simulink model "Simulacion_Trifasico_Fuzzy_v10_v12"  (R2024a)
settings: Solver=ode3  StartTime=0  StopTime=tend  FixedStep=0.01  RelTol=1e-3
values from neighbouring files (symbols this model uses):
  ts = 0.1    [Fuzzy_init.m]    (also in MPC_linealizar_v6.m)
libraries: simulink x6, eeStairGenerator x6, fuzblock x1
settings Model: Creator=Ivan  LastModifiedBy=Ivan
settings DebuggingCC: UnderSpecifiedDimensionMsg=warning
settings ConfigComp: PLC_TargetIDE=tiaportal  PLC_MultiTBSigbuilderTimeRange=off  PLC_FoldFBCallOutputVar=off  PLC_RemoveUnusedSSMethodCallArguments=off  PLC_UseCallOutputArgSyntax=off  PLC_EnableUnsignedAndDoubleTypes=off  PLC_EnableUDTSplitting=off  PLC_MaxFieldsInUDT=500  PLC_InlineEnumCastFunction=off

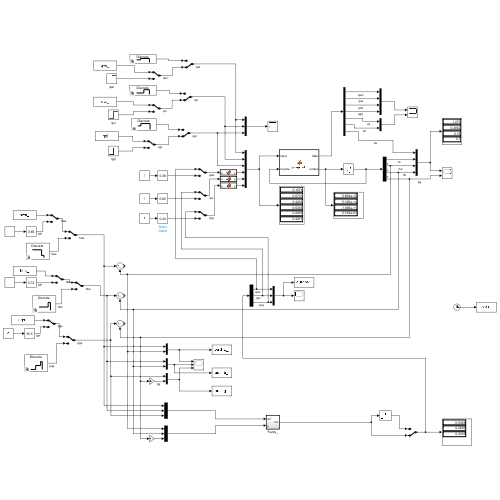
[thumbnail: Simulink's stored preview of the top-level diagram]
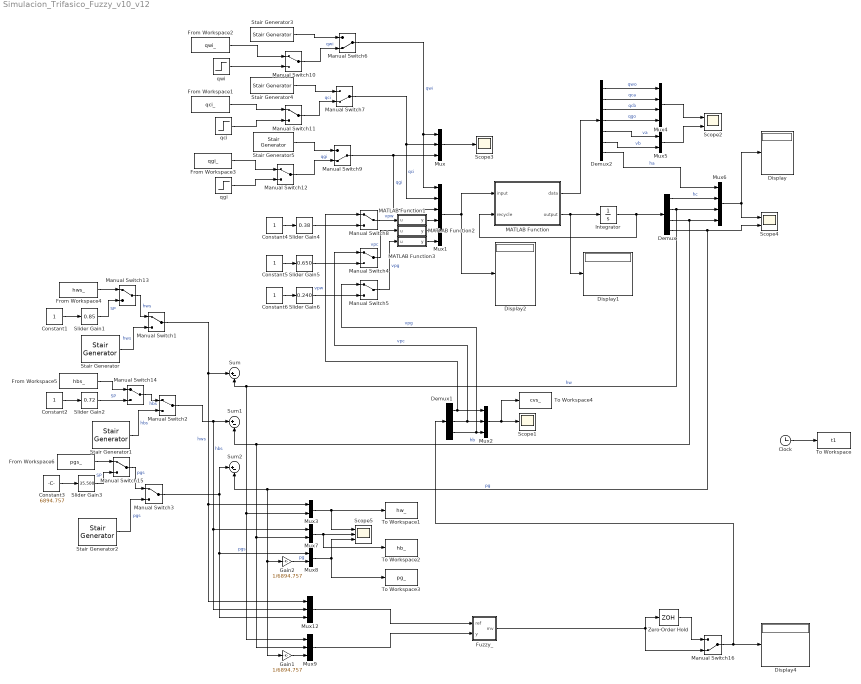
== system Simulacion_Trifasico_Fuzzy_v10_v12 ==
  Clock : Clock
  Constant{1..2,4..6} (5 alike) : Constant
  Constant3 : Constant  Value=6894.757
  Demux : Demux
  Demux1 : Demux  Outputs=3
  Demux2 : Demux  Outputs=7
  Display{,1..2,4} (4 alike) : Display
  From Workspace1 : FromWorkspace  VariableName=qci_  SampleTime=ts
  From Workspace2 : FromWorkspace  VariableName=qwi_  SampleTime=ts
  From Workspace3 : FromWorkspace  VariableName=qgi_  SampleTime=ts
  From Workspace4 : FromWorkspace  VariableName=hws_  SampleTime=ts
  From Workspace5 : FromWorkspace  VariableName=hbs_  SampleTime=ts
  From Workspace6 : FromWorkspace  VariableName=pgs_  SampleTime=ts
  Fuzzy_ : Subsystem  TreatAsAtomicUnit=on  SystemSampleTime=0.1
  Gain1 : Gain  Gain=1/6894.757
  Gain2 : Gain  Gain=1/6894.757
  Integrator : Integrator  InitialCondition=[0.4737; 0.80; 0.72; 37*6894.757]  LimitOutput=on  LowerSaturationLimit=0
  MATLAB Function : MATLAB Function  TreatAsAtomicUnit=on
  MATLAB Function1 : MATLAB Function  TreatAsAtomicUnit=on
  MATLAB Function2 : MATLAB Function  TreatAsAtomicUnit=on
  MATLAB Function3 : MATLAB Function  TreatAsAtomicUnit=on
  Manual Switch{1..5,8,10..15} (12 alike) : ManualSwitch
  Manual Switch{6..7,9,16} (4 alike) : ManualSwitch  CurrentSetting=0
  Mux{,2,9,12} (4 alike) : Mux  Inputs=3
  Mux1 : Mux  Inputs=6
  Mux{3,5,7..8} (4 alike) : Mux  Inputs=2
  Mux4 : Mux
  Mux6 : Mux
  Scope1 : Scope
  Scope2 : Scope  NumInputPorts=2
  Scope3 : Scope
  Scope4 : Scope  NumInputPorts=2
  Scope5 : Scope  NumInputPorts=3
  Slider Gain1 : simulink/Math Operations/Slider Gain  gain=0.85  low=0  high=1
  Slider Gain2 : simulink/Math Operations/Slider Gain  gain=0.72  low=0  high=1
  Slider Gain3 : simulink/Math Operations/Slider Gain  gain=35.500  low=0  high=50
  Slider Gain4 : simulink/Math Operations/Slider Gain  gain=0.38  low=0  high=1
  Slider Gain5 : simulink/Math Operations/Slider Gain  gain=0.650  low=0  high=1
  Slider Gain6 : simulink/Math Operations/Slider Gain  gain=0.240  low=0  high=1
  Stair Generator : eeStairGenerator/Stair Generator  LabelModeActiveChoice=Discrete  TimeInput=[0 2000 2500]  AmplitudeInput=[0.85 0.80 0.78]  SampleTime=0.01  RepeatPattern=off  OutDataTypeStr=double
      settings: LibrarySourceBlock=ee_sl_lib/General Control/Stair Generator
  Stair Generator1 : eeStairGenerator/Stair Generator  LabelModeActiveChoice=Discrete  TimeInput=[0 2250 2750]  AmplitudeInput=[0.72 0.75 0.70]  SampleTime=0.01  RepeatPattern=off  OutDataTypeStr=double
      settings: LibrarySourceBlock=ee_sl_lib/General Control/Stair Generator
  Stair Generator2 : eeStairGenerator/Stair Generator  LabelModeActiveChoice=Discrete  TimeInput="[0 1500 3000  3500]"  AmplitudeInput=[35 40 45 35]*6894.757  SampleTime=0.01  RepeatPattern=off  OutDataTypeStr=double
      settings: LibrarySourceBlock=ee_sl_lib/General Control/Stair Generator
  Stair Generator3 : eeStairGenerator/Stair Generator  LabelModeActiveChoice=Discrete  TimeInput=[0 1000 3250]  AmplitudeInput=[0.1374 0.1774 0.0474]  SampleTime=0.01  RepeatPattern=off  OutDataTypeStr=double
      settings: LibrarySourceBlock=ee_sl_lib/General Control/Stair Generator
  Stair Generator4 : eeStairGenerator/Stair Generator  LabelModeActiveChoice=Discrete  TimeInput=[0 1750 3100]  AmplitudeInput=[0.0711 0.1815 0.0298]  SampleTime=0.01  RepeatPattern=off  OutDataTypeStr=double
      settings: LibrarySourceBlock=ee_sl_lib/General Control/Stair Generator
  Stair Generator5 : eeStairGenerator/Stair Generator  LabelModeActiveChoice=Discrete  TimeInput=[0 1000 3750]  AmplitudeInput=[0.4906 0.79606 0.006]  SampleTime=0.01  RepeatPattern=off  OutDataTypeStr=double
      settings: LibrarySourceBlock=ee_sl_lib/General Control/Stair Generator
  Sum : Sum  Inputs=|+-
  Sum1 : Sum  Inputs=|+-
  Sum2 : Sum  Inputs=|+-
  To Workspace : ToWorkspace  VariableName=t1  SampleTime=0.1
  To Workspace1 : ToWorkspace  VariableName=hw_  SampleTime=0.1
  To Workspace2 : ToWorkspace  VariableName=hb_  SampleTime=0.1
  To Workspace3 : ToWorkspace  VariableName=pg_  SampleTime=0.1
  To Workspace4 : ToWorkspace  VariableName=cvs_  SampleTime=0.1
  Zero-Order Hold : ZeroOrderHold  SampleTime=-1
  qci : Step  After=.0711  SampleTime=0
  qgi : Step  After=.4906  SampleTime=0
  qwi : Step  After=.1374  SampleTime=0
  wires:
  Mux/1 -> Scope3/1
  Mux2/1 -> To Workspace4/1, Scope1/1
  Demux2/1 -> Mux4/1  "qwo"
  Demux2/2 -> Mux4/2  "qca"
  Demux2/3 -> Mux4/3  "qcb"
  Demux2/4 -> Mux4/4  "qgo"
  Demux2/5 -> Mux5/1  "va"
  Demux2/6 -> Mux5/2  "vb"
  Mux4/1 -> Scope2/1
  Mux5/1 -> Scope2/2
  Demux2/7 -> Mux6/1  "ha"
  Integrator/1 -> MATLAB Function/2(recycle), Demux/1
  Demux/1 -> Mux6/2  "hc"
  Demux/2 -> Mux9/1, Mux3/2, Sum/2, Mux6/3  "hw"
  Demux/3 -> Mux6/4, Mux9/2, Mux7/2, Sum1/2  "hb"
  Mux6/1 -> Display/1, Scope4/1
  Demux/4 -> Scope4/2, Gain1/1, Gain2/1, Sum2/2  "pg"
  Mux1/1 -> MATLAB Function/1(input), Display2/1
  MATLAB Function/2(output) -> Display1/1, Integrator/1
  MATLAB Function/1(data) -> Demux2/1
  Mux3/1 -> Scope5/1, To Workspace1/1
  Mux7/1 -> To Workspace2/1, Scope5/2
  Mux8/1 -> To Workspace3/1, Scope5/3
  Constant1/1 -> Slider Gain1/1
  Manual Switch1/1 -> Sum/1, Mux12/1, Mux3/1  "hws"
  Stair Generator/1 -> Manual Switch1/2  "hws"
  Constant2/1 -> Slider Gain2/1
  Manual Switch2/1 -> Mux7/1, Mux12/2, Sum1/1  "hbs"
  Constant3/1 -> Slider Gain3/1
  Manual Switch3/1 -> Sum2/1, Mux12/3, Mux8/1  "pgs"
  Stair Generator1/1 -> Manual Switch2/2  "hbs"
  Stair Generator2/1 -> Manual Switch3/2  "pgs"
  Constant4/1 -> Slider Gain4/1
  Slider Gain4/1 -> Manual Switch8/2
  Slider Gain5/1 -> Manual Switch4/2
  Constant5/1 -> Slider Gain5/1
  Slider Gain6/1 -> Manual Switch5/2
  Constant6/1 -> Slider Gain6/1
  Stair Generator3/1 -> Manual Switch6/1
  Stair Generator4/1 -> Manual Switch7/1
  Stair Generator5/1 -> Manual Switch9/1
  Manual Switch6/1 -> Mux1/1, Mux/1  "qwi"
  Manual Switch7/1 -> Mux/2, Mux1/2  "qci"
  Manual Switch9/1 -> Mux/3, Mux1/3  "qgi"
  Clock/1 -> To Workspace/1
  qwi/1 -> Manual Switch10/2
  Manual Switch10/1 -> Manual Switch6/2  "qwi"
  From Workspace2/1 -> Manual Switch10/1
  qci/1 -> Manual Switch11/2
  Manual Switch11/1 -> Manual Switch7/2  "qci"
  From Workspace1/1 -> Manual Switch11/1
  qgi/1 -> Manual Switch12/2
  Manual Switch12/1 -> Manual Switch9/2  "qgi"
  From Workspace3/1 -> Manual Switch12/1
  Slider Gain1/1 -> Manual Switch13/2  "SP"
  Manual Switch13/1 -> Manual Switch1/1  "hws"
  Slider Gain2/1 -> Manual Switch14/2  "SP"
  Manual Switch14/1 -> Manual Switch2/1  "hbs"
  Manual Switch15/1 -> Manual Switch3/1  "pgs"
  Slider Gain3/1 -> Manual Switch15/2  "SP"
  From Workspace4/1 -> Manual Switch13/1
  From Workspace5/1 -> Manual Switch14/1
  From Workspace6/1 -> Manual Switch15/1
  Manual Switch5/1 -> MATLAB Function3/1(u)  "vpg"
  Manual Switch4/1 -> MATLAB Function2/1(u)  "vpc"
  Manual Switch8/1 -> MATLAB Function1/1(u)  "vpw"
  MATLAB Function1/1(y) -> Mux1/4
  MATLAB Function2/1(y) -> Mux1/5
  MATLAB Function3/1(y) -> Mux1/6
  Gain1/1 -> Mux9/3
  Demux1/1 -> Manual Switch8/1, Mux2/1  "vpw"
  Demux1/2 -> Manual Switch4/1, Mux2/2  "vpc"
  Demux1/3 -> Mux2/3, Manual Switch5/1  "vpg"
  Gain2/1 -> Mux8/2  "pg"
  Zero-Order Hold/1 -> Manual Switch16/1
  Manual Switch16/1 -> Demux1/1, Display4/1
  Fuzzy_/1(mv) -> Manual Switch16/2, Zero-Order Hold/1
  Mux12/1 -> Fuzzy_/1(ref)
  Mux9/1 -> Fuzzy_/2(y)

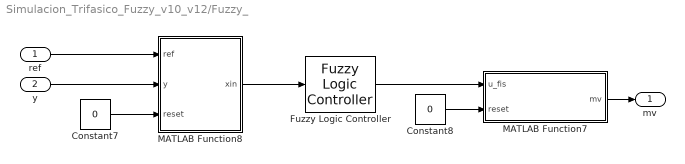
== system Simulacion_Trifasico_Fuzzy_v10_v12/Fuzzy_ ==
  ref : Inport
  y : Inport  Port=2
  Constant7 : Constant  Value=0
  Constant8 : Constant  Value=0
  Fuzzy Logic Controller : fuzblock/Fuzzy Logic  Controller  FIS=fis_tpsep_1block  OutputSampleNumber=101  DataType=double  FuzzifiedInputs=off  RuleFiringStrengths=off  RuleOutputs=off  AggregatedOutputs=off  SimulateUsing=Interpreted execution  OutOfRangeInputValueMessage=warning  NoRuleFiredMessage=warning  EmptyOutputFuzzySetMessage=warning
  MATLAB Function7 : MATLAB Function  TreatAsAtomicUnit=on
  MATLAB Function8 : MATLAB Function  TreatAsAtomicUnit=on
  mv : Outport
  wires:
  ref/1 -> MATLAB Function8/1(ref)
  Constant7/1 -> MATLAB Function8/3(reset)
  MATLAB Function8/1(xin) -> Fuzzy Logic Controller/1
  Fuzzy Logic Controller/1 -> MATLAB Function7/1(u_fis)
  Constant8/1 -> MATLAB Function7/2(reset)
  MATLAB Function7/1(mv) -> mv/1
  y/1 -> MATLAB Function8/2(y)

== matlab function Simulacion_Trifasico_Fuzzy_v10_v12/MATLAB Function ==
  data: input input size=6; data output size=7; output output size=4; recycle input size=4
function [data, output] = tpsep_v12(input, recycle)
%#codegen
% Codigo del bloque MATLAB Function de la planta, version corregida (tpsep_v12).
% crear_modelos_v12 copia este codigo dentro del bloque de cada modelo y cambia el nombre
% de la funcion para que coincida con el del bloque. Mismas entradas y salidas que el
% bloque original:
%   recycle = [hc hw hb pg]          (pg: presion MANOMETRICA en Pa)
%   input   = [qwi qci qgi vpw vpc vpg]  (qgi en condiciones estandar)
%   data    = [qwo; qca; qcb; qgo; va; vb; ha]
%   output  = [dhc; dhw; dhb; dpg]
% Correcciones (todas activas): balance de gas con presion absoluta, caudal de gas estandar
% convertido a condiciones del recipiente, una sola base de presiones, flujo critico en la
% valvula de gas, balance de la capa de crudo con V(Hw+Hc)-V(Hw) y colector que se vacia
% aunque no haya rebose.

qwi = input(1);
qci = input(2);
qgi = input(3);
vpw = min(max(input(4),0),1);
vpc = min(max(input(5),0),1);
vpg = min(max(input(6),0),1);

% Parametros (iguales a tpsep_v11)
ds   = 3.048;     % Diametro del separador            [m]
La   = 15.1724;   % Longitud de la camara              [m]
Lb   = 3.1076;    % Longitud del colector              [m]
hs   = 1.2192;    % Altura del vertedero               [m]
kvw  = 5.15e-4;   % Coef. valvula de agua
poa  = 101325;    % Presion aguas abajo v. agua (absoluta) [Pa]
kvc  = 7.15e-4;   % Coef. valvula de crudo
pob  = 101325;    % Presion aguas abajo v. crudo (absoluta) [Pa]
kvg  = 80.0;      % Coef. valvula de gas
poc  = 101325;    % Presion aguas abajo v. gas (absoluta) [Pa]
rhoc = 802.525;   % Densidad del crudo                 [kg/m^3]
sgc  = 0.9134;    % Gravedad especifica del crudo
rhow = 997.8;     % Densidad del agua                  [kg/m^3]
sgw  = 1.00;      % Gravedad especifica del agua
mgas = 28.04;     % Peso molecular del gas             [g/mol]
mair = 28.96;     % Peso molecular del aire            [g/mol]
g    = 9.81;      % Gravedad                           [m/s^2]
T    = 355.37;    % Temperatura del recipiente         [K]
Patm = 101325;    % Presion atmosferica                [Pa]
Pstd = 101325;    % Presion estandar (14.696 psia)     [Pa]
Tstd = 288.706;   % Temperatura estandar (60 F)        [K]
PA2PSI = 1.450377e-4;

% Estados
hc = max(min(recycle(1), hs-1e-6), 1e-6);
hw = max(min(recycle(2), hs-1e-6), 1e-6);
hb = max(min(recycle(3), 2.5), 1e-6);
pg = max(recycle(4), 1000);
pabs = pg + Patm;

vt = hemivolt(ds, La, Lb);
ha = hw + hc;

% Rebose sobre el vertedero
qca = 0;
if ha > hs
    H = max(ha - hs, 0);
    qca = 0.415*max(ds - 0.2*H, 0)*(H^1.5)*sqrt(2*g);
    if ~isfinite(qca) || qca < 0, qca = 0; end
end

% Valvulas de liquido, presiones absolutas
qcb = 0;
argcb = (pabs + rhoc*g*hb - pob)/sgc;
if argcb > 0, qcb = kvc*vpc*sqrt(argcb); end
if ~isfinite(qcb) || qcb < 0, qcb = 0; end

qwo = 0;
argwo = (pabs + rhoc*g*hc + rhow*g*hw - poa)/sgw;
if argwo > 0, qwo = kvw*vpw*sqrt(argwo); end
if ~isfinite(qwo) || qwo < 0, qwo = 0; end

% Valvula de gas (psia y grados Rankine), con flujo critico
Tf = (T - 273.15)*9/5 + 32;
TR = Tf + 460;
Gg = mgas/mair;
p1 = pabs*PA2PSI;
p2 = max(poc*PA2PSI, 0.5*p1);
dp2 = p1^2 - p2^2;
qgo = 0;
if dp2 > 0 && vpg > 0
    qgo = 962*kvg*vpg*sqrt(dp2/(Gg*TR))*7.86579e-6;   % m^3/s estandar
end
if ~isfinite(qgo) || qgo < 0, qgo = 0; end

% Volumenes
va = hemivols(min(max(ha,0),ds), La, ds);
vb = hemivols(min(max(hb,0),ds), Lb, ds);

% Balances de liquido
eps_h = 1e-4;
dhw = (qwi - qwo)/hemihead(max(hw,eps_h), ds, La);
dha = (qwi - qwo + qci - qca)/hemihead(max(min(ha, ds-eps_h), eps_h), ds, La);
dhc = dha - dhw;
dhb = (qca - qcb)/hemihead(max(hb,eps_h), ds, Lb);

% Balance de gas
Vgas = max(vt - va - vb, 1e-3);
qliq = qci + qwi - qwo - qcb;
dpg = (Pstd*T/Tstd*(qgi - qgo) + pabs*qliq)/Vgas;
if ~isfinite(dpg), dpg = 0; end

data   = [qwo; qca; qcb; qgo; va; vb; ha];
output = [dhc; dhw; dhb; dpg];
end

== matlab function Simulacion_Trifasico_Fuzzy_v10_v12/MATLAB Function1 ==
  data: u input; y output
function y = fcn(u)

% y = 1-tanh(u);
y = (u);

== matlab function Simulacion_Trifasico_Fuzzy_v10_v12/MATLAB Function2 ==
  data: u input; y output
function y = fcn(u)

% y = 1-tanh(u);
y = (u);

== matlab function Simulacion_Trifasico_Fuzzy_v10_v12/MATLAB Function3 ==
  data: u input; y output
function y = fcn(u)

% y = 1-tanh(u);
y = (u);

== matlab function Simulacion_Trifasico_Fuzzy_v10_v12/Fuzzy_/MATLAB Function8 ==
  settings: updateMethod=DISCRETE
  data: ref input; y input; xin output; reset input
function xin = Fuzzy_Preprocess(ref, y, reset)
% Preprocesamiento del controlador fuzzy MIMO (replica main_Fuzzy_2.m).
%
%   ref = [hw_sp; hb_sp; pg_sp]    y = [hw; hb; pg]
%   xin = [e_hw; de_hw; e_hb; de_hb; e_pg; de_pg]  -> FIS de 6 entradas
%
% Puerto reset: 0 = operacion normal, distinto de 0 = reinicia estados.
%#codegen

% ---------------- Escalas de entrada al FIS ----------------
%             hw     hb     pg
Ke  = [  0.30;  0.60;  0.09];    % escala del error
Kde = [ 22.00; 12.00;  3.00];    % escala de la derivada

% NOTA: en el lazo de gas Kde/Ke = 100, asi que el canal derivativo pesa
% mas que el del error (medido: 1.4x durante los transitorios). Es la
% entrada mas sensible al periodo real de ejecucion. Si reaparece el
% chattering de vpg, bajar Kde(3) de 6.0 a 2.0 es la correccion de fondo.

% ---------------- Estados persistentes ----------------
persistent e_ant initialized

if isempty(initialized) || reset ~= 0
    e_ant = zeros(3,1);
    initialized = true;
end

% ---------------- Error (PV - SP) ----------------
e = y(:) - ref(:);

% ---------------- Derivada discreta (por muestra) ----------------
de    = e - e_ant;
e_ant = e;

% ---------------- Escalamiento ----------------
xin = zeros(6,1);
xin(1) = e(1)*Ke(1);   xin(2) = de(1)*Kde(1);
xin(3) = e(2)*Ke(2);   xin(4) = de(2)*Kde(2);
xin(5) = e(3)*Ke(3);   xin(6) = de(3)*Kde(3);

% ---------------- Saturacion de las entradas del FIS ----------------
% DESACTIVADA para replicar el script: evalfis no satura, y si una entrada
% sale de [-1,1] ninguna MF dispara y el FIS devuelve el punto medio (0).
% El bloque Fuzzy Logic Controller y su codigo generado hacen lo mismo.
SAT_XIN = false;

if SAT_XIN
    for i = 1:6
        if xin(i) > 1.0
            xin(i) = 1.0;
        elseif xin(i) < -1.0
            xin(i) = -1.0;
        end
    end
end

end

== matlab function Simulacion_Trifasico_Fuzzy_v10_v12/Fuzzy_/MATLAB Function7 ==
  settings: updateMethod=DISCRETE
  data: u_fis input; reset input; mv output
function mv = Fuzzy_MV(u_fis, reset)
% Convierte las 3 salidas del FIS en aperturas de valvula.
%
%   u_fis = [u_vpw; u_vpc; u_vpg]   (salida del FIS, rango [-1,1])
%   mv    = [vpw;   vpc;   vpg  ]   saturadas en [0.01, 0.99]
%
% Debe ejecutarse a Ts = 0.1 s (subsistema Fuzzy_ con Sample time = 0.1).
%
%#codegen

% ---------------- Ganancias de integracion ----------------
% Valor original del script: Kcv = [1.5; 1.5; 1.5]
Kcv = [4.0; 2.5; 2.25];        % por muestra de 0.1 s

% ---------------- Limites de la apertura ----------------
MV_MIN = 0.01;
MV_MAX = 0.99;

cv0 = [MV_MIN; MV_MIN; MV_MIN];   % arranque desde el minimo, como el script

% ---------------- Limitador de velocidad (opcional) ----------------
% Desactivado por defecto para no alterar la respuesta validada.
% Poner en true si reaparece el chattering de vpg: recorta los saltos
% grandes (se midieron incrementos de hasta 0.154 en una sola ejecucion)
% sin afectar la dinamica lenta, cuyo percentil 99 es 0.0159.
RATE_ENABLE = true;
RATE_MAX    = [0.10; 0.10; 0.03];   % por muestra de 0.1 s

% ---------------- Estados persistentes ----------------
persistent cv cv_ant initialized

if isempty(initialized) || reset ~= 0
    cv     = cv0;
    cv_ant = cv0;
    initialized = true;
end

% ---------------- Integracion del mando difuso ----------------
cv = cv + Kcv .* u_fis(:);

% Anti-windup: el acumulador se limita al mismo rango que la apertura
for i = 1:3
    if cv(i) > MV_MAX
        cv(i) = MV_MAX;
    elseif cv(i) < MV_MIN
        cv(i) = MV_MIN;
    end
end

% ---------------- Limitador de velocidad ----------------
if RATE_ENABLE
    for i = 1:3
        d = cv(i) - cv_ant(i);
        if d > RATE_MAX(i)
            cv(i) = cv_ant(i) + RATE_MAX(i);
        elseif d < -RATE_MAX(i)
            cv(i) = cv_ant(i) - RATE_MAX(i);
        end
    end
end

cv_ant = cv;

% ---------------- Salida ----------------
mv = cv;

end
